simulink model "Controller_torque_cbf"  (R2026b)
settings: Solver=ode4  StopTime=Inf  FixedStep=1e-3
values from neighbouring files (symbols this model uses):
  Dn = 20 * ones(7,1)    [init_torque_cbf.m]
  H_0_cy = H_0_pr * H_pr_cy    [init_torque_cbf.m]
  H_home = getTransform(Franka_robot, q_home, 'panda_link8', 'panda_link0')    [init_torque_cbf.m]
  Kn = 0 * ones(7,1)    [init_torque_cbf.m]
  q_home = q_init    [init_torque_cbf.m]
  q_init = [0 0  0  -(2/4)*pi  0  pi/2  -pi/4]'    [init_torque_cbf.m]
undefined symbols (not defined in the file or in its folder): cbf_torque_params, DiscIntNeverNeededParam, Fext_mag, T_final, X, Y, Z
libraries: sm_lib x162, nesl_utility x44, matrix_library x3, Robotics_lib x1
(part 6 of 12)

== matlab function Controller_torque_cbf/Dynamic Parameters/Gravity Vector1 ==
  data: q_state input; g output
function g = Franka_Gravitational(q_state)
% Author: TU Wien, ACIN Robotics group
% Optimized and generated from Maple
  g = zeros(7,1);

  t30 = q_state(4);
  t20 = sin(t30);
  t25 = cos(t30);
  t29 = q_state(5);
  t24 = cos(t29);
  t50 = q_state(7);
  t41 = sin(t50);
  t42 = cos(t50);
  t12 = -0.7588510661394e-1 * t41 + 0.3068018192664e-1 * t42;
  t11 = 0.66581089427925e0 + t12;
  t19 = sin(t29);
  t47 = t11 * t19;
  t28 = q_state(6);
  t18 = sin(t28);
  t14 = 0.67524884163189e0 * t18;
  t51 = t14 - 0.14375311619778e0;
  t13 = 0.7588510661394e-1 * t42 + 0.3068018192664e-1 * t41;
  t10 = -0.161833169193795e1 - t13;
  t23 = cos(t28);
  t9 = t10 * t23;
  t7 = -t9 + t51;
  t3 = t7 * t24 - 0.48076874943165e1 - t47;
  t40 = 0.67524884163189e0 * t23;
  t48 = t10 * t18;
  t35 = t40 + t48;
  t5 = 0.1687990566084543e2 - t35;
  t54 = t20 * t3 + t25 * t5;
  t53 = -t20 * t5 + t25 * t3;
  t52 = t7 * t19;
  t46 = t11 * t24;
  t45 = t12 * t18;
  t44 = t12 * t23;
  t32 = q_state(2);
  t22 = sin(t32);
  t31 = q_state(3);
  t26 = cos(t31);
  t43 = t22 * t26;
  t38 = t13 * t19 + t24 * t44;
  t36 = 0.27690780075318e0 + t46;
  t33 = -0.1e1 * t9 + t51;
  t27 = cos(t32);
  t21 = sin(t31);
  t8 = t14 - t9;
  t1 = -0.671158958634432e1 - t53;
  g(6,1) = (((-0.1e1 * t48 - t40) * t24 * t25 + t8 * t20) * t26 + t35 * t21 * t19) * t22 + (t20 * t24 * t35 + t25 * t8) * t27;
  g(3,1) = (-t1 * t21 + (t36 + t52) * t26) * t22;
%   g(1,1) = 0.0e0;
  g(5,1) = (t46 + t52) * t25 * t43 + (-0.1e1 * t46 - 0.1e1 * t52) * t20 * t27 + (-0.1e1 * t47 + t33 * t24) * t22 * t21;
  g(2,1) = -0.1e1 * (0.3045357582685272e2 + t54) * t22 + (t1 * t26 + 0.1993386669246e-1 + (t19 * t33 + t36) * t21) * t27;
  g(4,1) = t27 * t53 + t43 * t54;
  g(7,1) = ((t20 * t45 - t25 * t38) * t26 + (-t13 * t24 + t19 * t44) * t21) * t22 + (t20 * t38 + t25 * t45) * t27;
  
end

== matlab function Controller_torque_cbf/Dynamic Parameters/MATLAB Function1 ==
  data: ROBOT input; M output; q input; dq input; C output; g output; Jg output; Jg_dot output; Htm output
function [M, C, g, Jg, Jg_dot, Htm] = DynamicMatrices(ROBOT, q, dq)
% UNTITLED Summary of this function goes here
%   Detailed explanation goes here
%     [xg, Htmb, M1, dM1, C1, g1, dg1, L1, dL1, J1, dJ1] = KaneScrew( ...
%     1, ROBOT.parent, ROBOT.g0, ROBOT.csi, ROBOT.com, ROBOT.Mass, ROBOT.S*q, ROBOT.S*dq );
% 
%     [M, dM] = deal( ROBOT.S.'*M1*ROBOT.S, ROBOT.S.'*dM1*ROBOT.S );
%     C = ROBOT.S.' * C1 * ROBOT.S;
%     [g, dg] = deal( ROBOT.S.'*g1, ROBOT.S.'*dg1 );
%     [L, dL] = deal( L1*ROBOT.S, dL1*ROBOT.S );
%     [Jb, dJb] = deal( J1*ROBOT.S, dJ1*ROBOT.S );
%     [Htm, J, dJ] = Kinematic(ROBOT.tcp, Htmb, Jb, dJb); 
%     [J_h, dJ_h] = Body2Hybrid( Htm, J, dJ, dq );



    

    [~, Htmb, M1, dM1, C1, g1, dg1, ~, ~, J1, dJ1] = KaneScrew( ...
    1, ROBOT.parent, ROBOT.g0, ROBOT.csi, ROBOT.com, ROBOT.Mass, ROBOT.S*q, ROBOT.S*dq );

    [M, ~] = deal( ROBOT.S.'*M1*ROBOT.S, ROBOT.S.'*dM1*ROBOT.S );
    C = ROBOT.S.' * C1 * ROBOT.S;
    [g, ~] = deal( ROBOT.S.'*g1, ROBOT.S.'*dg1 );
    [Jb, dJb] = deal( J1*ROBOT.S, dJ1*ROBOT.S );
    [Htm, J, dJ] = Kinematic(ROBOT.tcp, Htmb, Jb, dJb); 
    [Jg, Jg_dot] = Body2Hybrid( Htm, J, dJ, dq );

end

== matlab function Controller_torque_cbf/task space controller/nullspace damping ==
  data: q input; q_dot input; q_ref input; Kn input; tau_nullspace output; Dn input; Jg input; JgRightPseu input
function tau_nullspace = NullspaceDamping(q, q_dot, q_ref, Kn, Dn, Jg, JgRightPseu)
    Kn = diag(Kn);
    Dn = diag(Dn);
    tau_nullspace = (eye(7) - Jg'*JgRightPseu') * (-Dn*q_dot -Kn*(q-q_ref));
end

== matlab function Controller_torque_cbf/Visualisation/MATLAB Function4 ==
  data: x_ref input; p_ref output
function p_ref = fcn(x_ref)

p_ref = x_ref(1:3);

end

== matlab function Controller_torque_cbf/task space controller/Damping Desing Selection/MATLAB Function2 ==
  data: LQ input; K_d output; v_vec input; D_d output; xi_vec input
function [K_d, D_d] = fcn(LQ, v_vec, xi_vec)


d_vec = 2.*(xi_vec.*sqrt(v_vec));

K_d = LQ*diag(v_vec)*transpose(LQ);
K_d = (K_d + transpose(K_d))./2;

D_d = LQ*diag(d_vec)*transpose(LQ);
D_d = (D_d + transpose(D_d))./2;

end
